simulink model "mars_rover_arm"  (R2025a)
settings: Solver=ode23t  StartTime=0.0  StopTime=50  FixedStep=1e-4  MaxStep=0.1  RelTol=1e-3  AbsTol=1e-3  EnableMultiTasking=on
PostLoadFcn:
  | load mars_rover_arm_joint_traj
values from neighbouring files (symbols this model uses):
  X = matrix_wayp_tgts(:,1)    [mars_rover_arm_task_space.m]
  Y = matrix_wayp_tgts(:,2)    [mars_rover_arm_task_space.m]
  Z = matrix_wayp_tgts(:,3)    [mars_rover_arm_task_space.m]
undefined symbols (not defined in the file or in its folder): Control, eeConfig
libraries: sm_lib x10, nesl_utility x4, mars_rover_lib x2, slpidlib x1, robotcorelib x1
Description:
  | Mars Rover Manipulator Inverse Kinematic Analysis
  | Copyright 2022-2025 The MathWorks, Inc.
settings Model: Creator=The MathWorks, Inc.  LastModifiedBy=smiller
settings SolverCC: AutoScaleAbsTol=off  AlgebraicLoopSolver=TrustRegion
settings DataIOCC: LimitDataPoints=on  MaxDataPoints=10000  ReturnWorkspaceOutputs=off  SignalLoggingName=logsout_mars_rover_arm
settings OptimizationCC: ReuseModelBlockBuffer=off  LifeSpan=inf
settings DebuggingCC: AllowSymbolicDim=off  SFUnexpectedBacktrackingDiag=warning  SFNoUnconditionalDefaultTransitionDiag=warning  SFExecutionAtInitializationDiag=none  ArithmeticOperatorsInVariantConditions=warning
settings ModelReferenceCC: EnableRefExpFcnMdlSchedulingChecks=on
settings SFSimCC: SimUseLocalCustomCode=off  CustomCodeUndefinedFunction=UseInterfaceOnly
settings RTWCC: RTWUseLocalCustomCode=off  GPUComputeCapability=3.5  DLArmComputeVersion=19.05
settings CodeAppCC: StateflowObjectComments=on
settings GRTTargetCC: TargetLangStandard=C89/C90 (ANSI)
settings ConfigComp: CovMetricSettings=dw  CovSaveCumulativeToWorkspaceVar=on  CovSaveSingleToWorkspaceVar=on  CovExternalEMLEnable=off  CovSFcnEnable=off
settings SimscapeCC: SimscapeLogType=all  SimscapeLogSimulationStatistics=on  SimscapeLogName=simlog_mars_rover_arm  SimscapeLogDataHistory=10000.0
settings DiagnosticsConfigSet: SimMechanicsUnconnectedFramePorts=none  SimMechanicsUnconnectedGeometryPorts=none  SimMechanicsConflictingReferenceFrames=none
settings ExplorerConfigSet: InternalSimMechanicsExplorerSettings="<ExplorerConfiguration><canonicalview>default</canonicalview><AnimationSetting><BasePlaybackSpeed>1.0</BasePlaybackSpeed><PlaybackSpeedFactor>4.0</PlaybackSpeedFactor></AnimationSetting><TilePanel><TileInfo><Tiles Columns=\"1\" Count=\"1\" Rows=\"1\"><Column Weight=\"1\"/><Row Weight=\"1\"/><Tile Height=\"1\" Width=\"1\" X=\"0\" Y=\"0\"/></Tiles></TileInfo><SceneInfo><SceneViewer><BGColor><R>1</R><G>1</G><B>1</B></BGColor><Camera><DoPerspective>off</DoPerspective><Position><X>56.6808179244821559</X><Y>33.5975972194638786</Y><Z>4.08245151996706923</Z></Position><Center><X>55.3334925254172916</X><Y>34.9449226185287358</Y><Z>2.73512612090218354</Z></Center><Up><X>-0.408248290463863073</X><Y>0.408248290463863073</Y><Z>0.816496580927726145</Z></Up><ViewLimDist>1</ViewLimDist><YLim>1.51407154321670534</YLim><XLim>3.3330786862056021</XLim></Camera></SceneViewer></SceneInfo></TilePanel><MechEditorPanel><Cameras/><GfxPanelCameraMap/><VideoCreator><PlaybackSpeedRatio>1.0</PlaybackSpeedRatio><FrameRate>30</FrameRate><VideoFormat>Motion JPEG AVI</VideoFormat><FrameSize>auto</FrameSize></VideoCreator></MechEditorPanel></ExplorerConfiguration>"

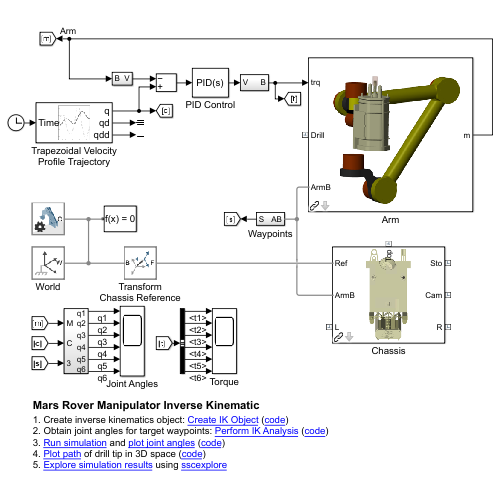
[thumbnail: Simulink's stored preview of the top-level diagram]
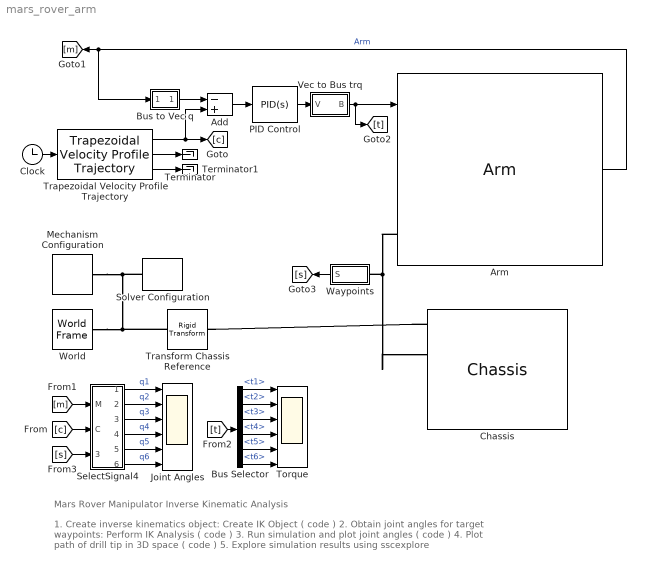
== system mars_rover_arm ==
  note: Mars Rover Manipulator Inverse Kinematic Analysis
  note: 1. Create inverse kinematics object: Create IK Object ( code )
      | 2. Obtain joint angles for target waypoints: Perform IK Analysis ( code )
      | 3. Run simulation and plot joint angles ( code )
      | 4. Plot path of drill tip in 3D space ( code )
      | 5. Explore simulation results using sscexplore
  Add : Sum  Inputs=-+
  Arm : mars_rover_lib/Arm  arm_q0_deg=arm_q0
  Bus Selector : BusSelector  OutputSignals=t1,t2,t3,t4,t5,t6
  Bus to Vec q : Subsystem
  Chassis : mars_rover_lib/Chassis  body_opc=0.2
  Clock : Clock
  Joint Angles : Scope  NumInputPorts=6
      settings: Title=Joint 1  ActiveDisplayYMinimum=-14.91429  ActiveDisplayYMaximum=110.52107  YLabel=Joint Angle (deg)
  Mechanism Configuration : sm_lib/Utilities/Mechanism Configuration  UniformGravity=Constant  GravityVector=[0 0 -3.81 ]  GravityVectorUnits=m/s^2  LinearizationDelta=0.001  JointModeTransitionNonlinearIterations=2
  PID Control : slpidlib/PID Controller  Controller=PID  Form=Parallel  TimeDomain=Continuous-time  UseExternalTs=off  SampleTime=-1  IntegratorMethod=Forward Euler  FilterMethod=Forward Euler  ControllerParametersSource=internal  P=Control.Arm.Kp  I=Control.Arm.Ki  UseKiTs=off  D=Control.Arm.Kd  UseExternalDerivativeSource=off  N=Control.Arm.N  UseFilter=on  TunerSelectOption=Transfer Function Based (PID Tuner App)  InitialConditionSource=internal  InitialConditionForIntegrator=0  InitialConditionForFilter=0  DifferentiatorICPrevScaledInput=0  ExternalReset=none  TrackingMode=off  Kt=1  LimitOutput=off  SatLimitsSource=internal  UpperSaturationLimit=inf  LowerSaturationLimit=-inf  LinearizeAsGain=on  AntiWindupMode=none  Kb=1  LimitIntegrator=off  UpperIntegratorSaturationLimit=inf  LowerIntegratorSaturationLimit=-inf  POutMin=[]  POutMax=[]  IOutMin=[]  IOutMax=[]  DOutMin=[]  DOutMax=[]  NOutMin=[]  NOutMax=[]  SumOutMin=[]  SumOutMax=[]  SaturationOutMin=[]  SaturationOutMax=[]  PParamMin=[]  PParamMax=[]  IParamMin=[]  IParamMax=[]  DParamMin=[]  DParamMax=[]  NParamMin=[]  NParamMax=[]  KbParamMin=[]  KbParamMax=[]  KtParamMin=[]  KtParamMax=[]  KbOutMin=[]  KbOutMax=[]  KtOutMin=[]  KtOutMax=[]  IntegratorOutMin=[]  IntegratorOutMax=[]  FilterOutMin=[]  FilterOutMax=[]  SumI1OutMin=[]  SumI1OutMax=[]  SumI2OutMin=[]  SumI2OutMax=[]  SumI3OutMin=[]  SumI3OutMax=[]  SumI4OutMin=[]  SumI4OutMax=[]  SumDOutMin=[]  SumDOutMax=[]  DifferentiatorOutMin=[]  DifferentiatorOutMax=[]  FilterDiffOutCoefMin=[]  FilterDiffOutCoefMax=[]  ReciprocalOutMin=[]  ReciprocalOutMax=[]  SumDenOutMin=[]  SumDenOutMax=[]  SumNumOutMin=[]  SumNumOutMax=[]  DivideOutMin=[]  DivideOutMax=[]  UdiffTsProdOutMin=[]  UdiffTsProdOutMax=[]  NTsProdOutMin=[]  NTsProdOutMax=[]  UintegralTsProdOutMin=[]  UintegralTsProdOutMax=[]  UngainTsProdOutMin=[]  UngainTsProdOutMax=[]  ClampingZeroOutDataTypeStr=Inherit: Inherit via back propagation  ClampingZeroOutMin=[]  ClampingZeroOutMax=[]  FilterDenConstantOutDataTypeStr=Inherit: Inherit via back propagation  FilterDenConstantOutMin=[]  FilterDenConstantOutMax=[]  PCopyOutDataTypeStr=Inherit: Inherit via back propagation  PCopyOutMin=[]  PCopyOutMax=[]  NCopyOutDataTypeStr=Inherit: Inherit via back propagation  NCopyOutMin=[]  NCopyOutMax=[]  IntegratorContinuousStateAttributes=''  IntegratorStateMustResolveToSignalObject=off  IntegratorRTWStateStorageClass=Auto  FilterContinuousStateAttributes=''  FilterStateMustResolveToSignalObject=off  FilterRTWStateStorageClass=Auto  ParallelPVariant=InternalParameters  IdealPVariant=Disabled  IVariant=InternalParameters  DVariant=InternalParameters  IntegratorVariant=Continuous  SatVariant=Disabled  AWVariant=Passthrough  PCopyVariant=Disabled  TRVariant=Disabled  FdbkBlocksVariant=Forward  IdealPFdbkVariant=Disabled  SatFdbkVariant=Disabled  DerivativeFilterVariant=ContFilter  NVariant=InternalParameters  NCopyVariant=Disabled  FilterICVariant=InternalICsFilter  IntegratorICVariant=InternalICs  ExternalResetVariant=Disabled  TRSumVariant=Passthrough  SumFdbkVariant=Disabled  SumVariant=Sum_PID  TsampFilterVariant=InternalTs  TsampNgainVariant=Passthrough  TsampIntegralVariant=Disabled_SignalSpec  ExternalSaturationOutDataTypeStr=Inherit: Same as second input  DerivativeSourceVariant=ErrorSignal  PreIntVariant=InternalPreInt
  SelectSignal4 : Subsystem
  Solver Configuration : nesl_utility/Solver Configuration  PhysicalDomain=network_engine_domain  SubClassName=solver  LeftPortType=input  RightPortType=generic  Tones=[]  Harmonics=[]  SimulateNoise=off  Profile=off  UseLocalSampling=off  EnableSwitchedLinearOptims=on  FrequencyDomain=off  UseCCode=off  RelTol=0.001  AbsTol=1e-06  MinStep=1e-09  ToWorkspace=off  RevertToSquareIcSolve=off  NumHomotopyIterations=100  PhasorMode=off  PhasorModeNumHarmonics=1  ConsistencySolver=NEWTON_FTOL  IndexReductionMethod=DerivativeReplacement  DoDC=off  ResidualTolerance=1e-09  ConsistencyTolSource=GLOBAL  ConsistencyAbsTol=0.001  ConsistencyRelTol=0.001  ConsistencyTolFactor=0.001  UseLocalSolver=off  LocalSolverChoice=NE_BACKWARD_EULER_ADVANCER  ResolveIndetEquations=on  FunctionEvalNumThread=1  LocalSolverSampleTime=0.001  DoFixedCost=off  MaxNonlinIter=3  MaxModeIter=2  ComputeImpulses=off  ImpulseIterations=2  LinearAlgebra=Sparse  LinearAlgebraNumThread=0  EquationFormulation=NE_TIME_EF  DelaysMemoryBudget=1024  AutomaticFiltering=on  FilteringTimeConstant=0.001  PartitionStorageMethod=AS_NEEDED  PartitionMemoryBudget=1024  PartitionMethod=FAST  MultibodyUseLocalSolver=off  MultibodyLocalSolverChoice=ODE1  MultibodyLocalSolverSampleTime=0.001
  Terminator : Terminator
  Terminator1 : Terminator
  Torque : Scope  NumInputPorts=6
      settings: Title=Joint 1  ActiveDisplayYMinimum=-72.39496  ActiveDisplayYMaximum=72.83074  YLabel=Torque (N*m)  DataLoggingVariableName=ScopeData2
  Transform Chassis Reference : sm_lib/Frames and Transforms/Rigid Transform  RotationMethod=None  FollAlignAxisA=+X  BaseAlignAxisA=+Y  FollAlignAxisB=+Y  BaseAlignAxisB=+Z  RotationStandardAxis=+X  RotationAngle=90  RotationAngleUnits=deg  RotationArbitraryAxis=[0 0 1]  RotationSequenceAxes=FollowerAxes  RotationSequence=XYX  RotationSequenceAngles=[0 0 0]  RotationSequenceAnglesUnits=deg  RotationMatrix=[1 0 0; 0 1 0; 0 0 1]  Quaternion=[1 0 0 0]  TranslationMethod=Cartesian  TranslationCartesianOffset=[55 35 2.8]  TranslationCartesianOffsetUnits=m  TranslationStandardAxis=+Z  TranslationStandardOffset=1.85  TranslationStandardOffsetUnits=m  TranslationROffset=0  TranslationROffsetUnits=m  TranslationThetaOffset=0  TranslationThetaOffsetUnits=deg  TranslationZOffset=0  TranslationZOffsetUnits=m
  Trapezoidal Velocity Profile Trajectory : robotcorelib/Trapezoidal Velocity Profile Trajectory  WaypointSource=Internal  Waypoints=arm_joint_traj'  NumParams=1  Parameter1=End Time  Parameter2=End Time  ParameterSource=Internal  PeakVelocity=[ 2; 2 ]  Acceleration=[ 1; 2 ]  EndTime=5  AccelTime=[ 1; 2 ]  SimulateUsing=Code generation
  Vec to Bus trq : Subsystem
  Waypoints : Subsystem
  World : sm_lib/Frames and Transforms/World Frame
  wires:
  Trapezoidal Velocity Profile Trajectory/1 -> [c], Add/2
  Clock/1 -> Trapezoidal Velocity Profile Trajectory/1
  Add/1 -> PID Control/1
  Bus to Vec q/1(V) -> Add/1
  Arm/1 -> Bus to Vec q/1(B), [m]  "Arm"
  PID Control/1 -> Vec to Bus trq/1(V)
  Vec to Bus trq/1(B) -> [t], Arm/1
  Trapezoidal Velocity Profile Trajectory/2 -> Terminator/1
  Trapezoidal Velocity Profile Trajectory/3 -> Terminator1/1
  SelectSignal4/4(q4) -> Joint Angles/4  "q4"
  SelectSignal4/1(q1) -> Joint Angles/1  "q1"
  SelectSignal4/6(q6) -> Joint Angles/6  "q6"
  SelectSignal4/3(q3) -> Joint Angles/3  "q3"
  SelectSignal4/2(q2) -> Joint Angles/2  "q2"
  SelectSignal4/5(q5) -> Joint Angles/5  "q5"
  [c] -> SelectSignal4/2(C)
  [m] -> SelectSignal4/1(M)
  [t] -> Bus Selector/1
  Bus Selector/1 -> Torque/1  "<t1>"
  Bus Selector/2 -> Torque/2  "<t2>"
  Bus Selector/3 -> Torque/3  "<t3>"
  Bus Selector/4 -> Torque/4  "<t4>"
  Bus Selector/5 -> Torque/5  "<t5>"
  Bus Selector/6 -> Torque/6  "<t6>"
  Waypoints/1(S) -> [s]
  [s] -> SelectSignal4/3(In3)
  connections:
  Mechanism Configuration/RConn1 -- World/RConn1 -- Transform Chassis Reference/LConn1 -- Solver Configuration/RConn1
  Chassis/LConn1 -- Transform Chassis Reference/RConn1
  Waypoints/LConn1 -- Chassis/LConn2 -- Arm/LConn2

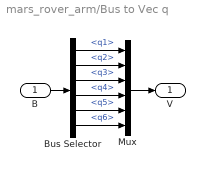
== system mars_rover_arm/Bus to Vec q ==
  B : Inport
  Bus Selector : BusSelector  OutputSignals=q.q1,q.q2,q.q3,q.q4,q.q5,q.q6
  Mux : Mux  Inputs=6
  V : Outport
  wires:
  Bus Selector/6 -> Mux/6  "<q6>"
  Bus Selector/4 -> Mux/4  "<q4>"
  Mux/1 -> V/1
  B/1 -> Bus Selector/1
  Bus Selector/1 -> Mux/1  "<q1>"
  Bus Selector/3 -> Mux/3  "<q3>"
  Bus Selector/2 -> Mux/2  "<q2>"
  Bus Selector/5 -> Mux/5  "<q5>"

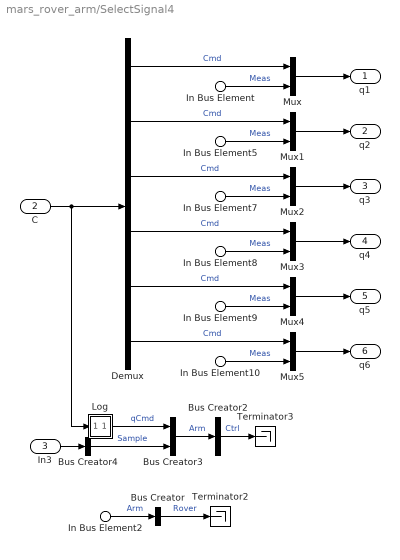
== system mars_rover_arm/SelectSignal4 ==
  In Bus Element2 : Inport  PortName=M
  In Bus Element : Inport  PortName=M  Element=q.q1
  In Bus Element5 : Inport  PortName=M  Element=q.q2
  In Bus Element7 : Inport  PortName=M  Element=q.q3
  In Bus Element8 : Inport  PortName=M  Element=q.q4
  In Bus Element9 : Inport  PortName=M  Element=q.q5
  In Bus Element10 : Inport  PortName=M  Element=q.q6
  C : Inport  Port=2
  In3 : Inport  Port=3
  Bus Creator : BusCreator  Inputs=1
  Bus Creator2 : BusCreator  Inputs=1
  Bus Creator3 : BusCreator  Inputs=2
  Bus Creator4 : BusCreator  Inputs=1
  Demux : Demux  Outputs=6
  "Log " : Subsystem
  Mux{,1..5} (6 alike) : Mux  Inputs=2
  Terminator2 : Terminator
  Terminator3 : Terminator
  q1 : Outport
  q2 : Outport  Port=2
  q3 : Outport  Port=3
  q4 : Outport  Port=4
  q5 : Outport  Port=5
  q6 : Outport  Port=6
  wires:
  In Bus Element10/1 -> Mux5/2  "Meas"
  Mux5/1 -> q6/1
  Demux/6 -> Mux5/1  "Cmd"
  Demux/5 -> Mux4/1  "Cmd"
  Mux4/1 -> q5/1
  In Bus Element9/1 -> Mux4/2  "Meas"
  In Bus Element8/1 -> Mux3/2  "Meas"
  Mux3/1 -> q4/1
  Demux/4 -> Mux3/1  "Cmd"
  Demux/3 -> Mux2/1  "Cmd"
  Mux2/1 -> q3/1
  Mux1/1 -> q2/1
  Demux/2 -> Mux1/1  "Cmd"
  Demux/1 -> Mux/1  "Cmd"
  Mux/1 -> q1/1
  In Bus Element/1 -> Mux/2  "Meas"
  In Bus Element5/1 -> Mux1/2  "Meas"
  In Bus Element7/1 -> Mux2/2  "Meas"
  C/1 -> "Log "/1(C), Demux/1
  Bus Creator/1 -> Terminator2/1  "Rover"
  In Bus Element2/1 -> Bus Creator/1  "Arm"
  Bus Creator2/1 -> Terminator3/1  "Ctrl"
  "Log "/1(A) -> Bus Creator3/1  "qCmd"
  In3/1 -> Bus Creator4/1
  Bus Creator3/1 -> Bus Creator2/1  "Arm"
  Bus Creator4/1 -> Bus Creator3/2  "Sample"

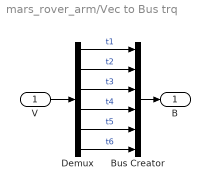
== system mars_rover_arm/Vec to Bus trq ==
  V : Inport
  Bus Creator : BusCreator  Inputs=6
  Demux : Demux  Outputs=6
  B : Outport
  wires:
  Demux/5 -> Bus Creator/5  "t5"
  Demux/2 -> Bus Creator/2  "t2"
  Demux/6 -> Bus Creator/6  "t6"
  Demux/1 -> Bus Creator/1  "t1"
  Demux/4 -> Bus Creator/4  "t4"
  V/1 -> Demux/1
  Bus Creator/1 -> B/1
  Demux/3 -> Bus Creator/3  "t3"

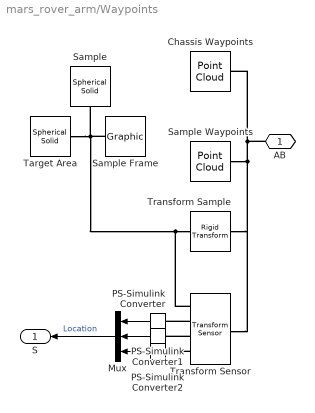
== system mars_rover_arm/Waypoints ==
  Chassis Waypoints : sm_lib/Curves and Surfaces/Point Cloud  CoordinatesMatrix=eeConfig.Targets{[1 2 5 6 7],1:3}  CoordinatesMatrixUnits=m  GraphicType=MarkerCloud  GraphicSphereRadius=5e-2  GraphicSphereRadiusUnits=m  GraphicVisPropType=SimpleVisualProperties  GraphicDiffuseColor=[0.302 0.7451 0.9333]  GraphicOpacity=0.5  GraphicSpecularColor=[0.5 0.5 0.5 1.0]  GraphicAmbientColor=[0.15 0.15 0.15 1.0]  GraphicEmissiveColor=[0.0 0.0 0.0 1.0]  GraphicShininess=75
  Mux : Mux  Inputs=3
  PS-Simulink Converter : nesl_utility/PS-Simulink Converter  PhysicalDomain=network_engine_domain  SubClassName=ps_output  LeftPortType=input  RightPortType=output  PseudoPeriodic=off  Frequencies=[]  VectorFormat=1-D array  Unit=inherit  AffineConversion=off
  PS-Simulink Converter1 : nesl_utility/PS-Simulink Converter  PhysicalDomain=network_engine_domain  SubClassName=ps_output  LeftPortType=input  RightPortType=output  PseudoPeriodic=off  Frequencies=[]  VectorFormat=1-D array  Unit=inherit  AffineConversion=off
  PS-Simulink Converter2 : nesl_utility/PS-Simulink Converter  PhysicalDomain=network_engine_domain  SubClassName=ps_output  LeftPortType=input  RightPortType=output  PseudoPeriodic=off  Frequencies=[]  VectorFormat=1-D array  Unit=inherit  AffineConversion=off
  Sample : sm_lib/Body Elements/Spherical Solid  SphereRadius=0.02  SphereRadiusUnits=m  ExportEntireGeometry=off  InertiaType=CalculateFromGeometry  BasedOnType=Mass  Density=1000  DensityUnits=kg/m^3  Mass=0.001  MassUnits=kg  CenterOfMass=[0 0 0]  CenterOfMassUnits=m  MomentsOfInertia=[1 1 1]  MomentsOfInertiaUnits=kg*m^2  ProductsOfInertia=[0 0 0]  ProductsOfInertiaUnits=kg*m^2  GraphicType=FromGeometry  MarkerShape=Sphere  MarkerSize=10  GraphicVisPropType=AdvancedVisualProperties  GraphicDiffuseColor=[1 0 0]  GraphicOpacity=1.0  GraphicSpecularColor=[0.5 0.5 0.5 1.0]  GraphicAmbientColor=[0.15 0.15 0.15 1.0]  GraphicEmissiveColor=[0.0 0.0 0.0 1.0]  GraphicShininess=25  DoExposeReferenceFrame=on  SerializedFrames=<Frames/>
  Sample Frame : sm_lib/Body Elements/Graphic  GraphicType=Marker  MarkerShape=Frame  MarkerSize=5  GraphicVisPropType=SimpleVisualProperties  GraphicDiffuseColor=[1 0 0]  GraphicOpacity=1.0  GraphicSpecularColor=[0.5 0.5 0.5 1.0]  GraphicAmbientColor=[0.15 0.15 0.15 1.0]  GraphicEmissiveColor=[0.0 0.0 0.0 1.0]  GraphicShininess=75
  Sample Waypoints : sm_lib/Curves and Surfaces/Point Cloud  CoordinatesMatrix=eeConfig.Targets{[3 4],1:3}  CoordinatesMatrixUnits=m  GraphicType=MarkerCloud  GraphicSphereRadius=5e-2  GraphicSphereRadiusUnits=m  GraphicVisPropType=SimpleVisualProperties  GraphicDiffuseColor=[0.4667 0.6745 0.1882]  GraphicOpacity=0.5  GraphicSpecularColor=[0.5 0.5 0.5 1.0]  GraphicAmbientColor=[0.15 0.15 0.15 1.0]  GraphicEmissiveColor=[0.0 0.0 0.0 1.0]  GraphicShininess=75
  Target Area : sm_lib/Body Elements/Spherical Solid  SphereRadius=0.35/4  SphereRadiusUnits=m  ExportEntireGeometry=off  InertiaType=CalculateFromGeometry  BasedOnType=Density  Density=1000  DensityUnits=kg/m^3  Mass=1  MassUnits=kg  CenterOfMass=[0 0 0]  CenterOfMassUnits=m  MomentsOfInertia=[1 1 1]  MomentsOfInertiaUnits=kg*m^2  ProductsOfInertia=[0 0 0]  ProductsOfInertiaUnits=kg*m^2  GraphicType=FromGeometry  MarkerShape=Sphere  MarkerSize=10  GraphicVisPropType=SimpleVisualProperties  GraphicDiffuseColor=[0.4 1.0 0.2]  GraphicOpacity=0.8  GraphicSpecularColor=[0.5 0.5 0.5 1.0]  GraphicAmbientColor=[0.15 0.15 0.15 1.0]  GraphicEmissiveColor=[0.0 0.0 0.0 1.0]  GraphicShininess=75  DoExposeReferenceFrame=on  SerializedFrames=<Frames/>
  Transform Sample : sm_lib/Frames and Transforms/Rigid Transform  RotationMethod=None  FollAlignAxisA=+X  BaseAlignAxisA=+Y  FollAlignAxisB=+Y  BaseAlignAxisB=+Z  RotationStandardAxis=+Z  RotationAngle=0.0  RotationAngleUnits=deg  RotationArbitraryAxis=[0 0 1]  RotationSequenceAxes=FollowerAxes  RotationSequence=XYX  RotationSequenceAngles=[0 0 0]  RotationSequenceAnglesUnits=deg  RotationMatrix=[1 0 0; 0 1 0; 0 0 1]  Quaternion=[1 0 0 0]  TranslationMethod=Cartesian  TranslationCartesianOffset=eeConfig.Targets{3,1:3}  TranslationCartesianOffsetUnits=m  TranslationStandardAxis=+Z  TranslationStandardOffset=0  TranslationStandardOffsetUnits=m  TranslationROffset=0  TranslationROffsetUnits=m  TranslationThetaOffset=0  TranslationThetaOffsetUnits=deg  TranslationZOffset=0  TranslationZOffsetUnits=m
  Transform Sensor : sm_lib/Frames and Transforms/Transform Sensor  MeasurementFrame=Base  RotationSequence=XYX  SenseAngle=off  SenseAxis=off  SenseQ=off  SenseR=off  SenseRotationSequence=off  SenseOmegaX=off  SenseOmegaY=off  SenseOmegaZ=off  SenseOmega=off  SenseQDot=off  SenseRDot=off  SenseRotationSequenceDot=off  SenseAlphaX=off  SenseAlphaY=off  SenseAlphaZ=off  SenseAlpha=off  SenseQDDot=off  SenseRDDot=off  SenseX=on  SenseY=on  SenseZ=on  SenseXYZ=off  SenseRad=off  SenseAzim=off  SenseDist=off  SenseInc=off  SenseXDot=off  SenseYDot=off  SenseZDot=off  SenseXYZDot=off  SenseRadDot=off  SenseAzimDot=off  SenseDistDot=off  SenseIncDot=off  SenseXDDot=off  SenseYDDot=off  SenseZDDot=off  SenseXYZDDot=off  SenseRadDDot=off  SenseAzimDDot=off  SenseDistDDot=off  SenseIncDDot=off
  AB : PMIOPort  Side=Left
  S : Outport
  wires:
  PS-Simulink Converter/1 -> Mux/1
  PS-Simulink Converter1/1 -> Mux/2
  PS-Simulink Converter2/1 -> Mux/3
  Mux/1 -> S/1  "Location"
  connections:
  AB/RConn1 -- Transform Sample/LConn1 -- Transform Sensor/LConn1 -- Sample Waypoints/LConn1 -- Chassis Waypoints/LConn1
  Target Area/RConn1 -- Transform Sensor/RConn1 -- Transform Sample/RConn1 -- Sample/RConn1 -- Sample Frame/RConn1
  Transform Sensor/RConn2 -- PS-Simulink Converter/LConn1
  Transform Sensor/RConn3 -- PS-Simulink Converter1/LConn1
  Transform Sensor/RConn4 -- PS-Simulink Converter2/LConn1

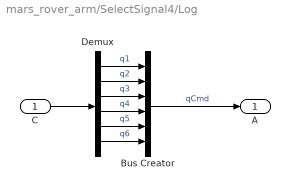
== system mars_rover_arm/SelectSignal4/Log  ==
  C : Inport
  Bus Creator : BusCreator  Inputs=6
  Demux : Demux  Outputs=6
  A : Outport
  wires:
  C/1 -> Demux/1
  Demux/1 -> Bus Creator/1  "q1"
  Demux/2 -> Bus Creator/2  "q2"
  Demux/3 -> Bus Creator/3  "q3"
  Demux/4 -> Bus Creator/4  "q4"
  Demux/5 -> Bus Creator/5  "q5"
  Demux/6 -> Bus Creator/6  "q6"
  Bus Creator/1 -> A/1  "qCmd"
